simulink model "FSI_2DOF_SS_TF_Simulink"  (R2021a)
settings: Solver=FixedStepAuto  StartTime=0.0  StopTime=5  FixedStep=1e-4  RelTol=1e-3  EnableMultiTasking=on
undefined symbols (not defined in the file): A2, B2, bias_1, bias_2, C2, D2, den_2DOF_1, den_2DOF_2, F_1, F_2, is_1, is_2, num_2DOF_1, num_2DOF_2, omega_1, omega_2, phase_1, phase_2, t_1, t_2, v_10, v_20, x_10, x_20
settings Model: Creator=FilipKsica  LastModifiedBy=FilipKsica
settings SolverCC: AlgebraicLoopSolver=TrustRegion
settings DataIOCC: LimitDataPoints=on  ReturnWorkspaceOutputs=off
settings OptimizationCC: LifeSpan=inf
settings DebuggingCC: AllowSymbolicDim=off  SFUnexpectedBacktrackingDiag=warning  SFNoUnconditionalDefaultTransitionDiag=warning  SFExecutionAtInitializationDiag=none  SFMachineParentedDataDiag=warning  ArithmeticOperatorsInVariantConditions=warning
settings ModelReferenceCC: PropagateSignalLabelsOutOfModel=off
settings SFSimCC: SimUseLocalCustomCode=off  CustomCodeUndefinedFunction=UseInterfaceOnly
settings RTWCC: RTWUseLocalCustomCode=off
settings CodeAppCC: StateflowObjectComments=on
settings GRTTargetCC: TargetLangStandard=C89/C90 (ANSI)
settings ConfigComp: CovMetricSettings=dw  CovSaveCumulativeToWorkspaceVar=on  CovSaveSingleToWorkspaceVar=on  CovExternalEMLEnable=off

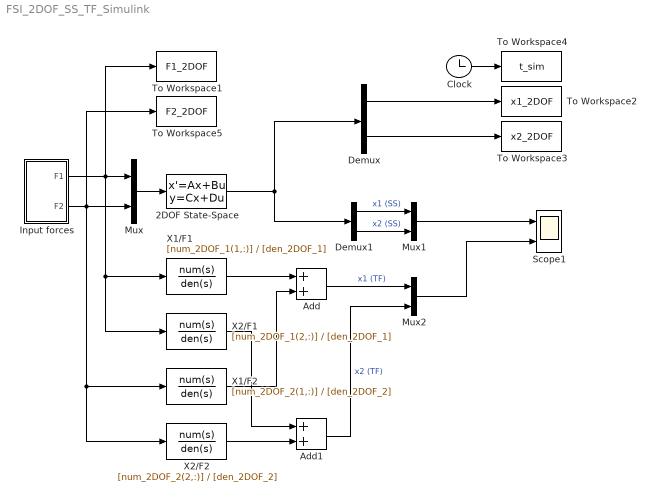
== system FSI_2DOF_SS_TF_Simulink ==
  2DOF State-Space : StateSpace  A=A2  B=B2  C=C2  D=D2  InitialCondition=[x_10 v_10 x_20 v_20]
  Add : Sum
  Add1 : Sum
  Clock : Clock
  Demux : Demux  Outputs=2
  Demux1 : Demux  Outputs=2
  Input forces : Subsystem
  Mux : Mux  Inputs=2
  Mux1 : Mux  Inputs=2
  Mux2 : Mux  Inputs=2
  Scope1 : Scope  NumInputPorts=2
  To Workspace1 : ToWorkspace  VariableName=F1_2DOF  SampleTime=-1
  To Workspace2 : ToWorkspace  VariableName=x1_2DOF  SampleTime=-1
  To Workspace3 : ToWorkspace  VariableName=x2_2DOF  SampleTime=-1
  To Workspace4 : ToWorkspace  VariableName=t_sim  SampleTime=-1
  To Workspace5 : ToWorkspace  VariableName=F2_2DOF  SampleTime=-1
  X1/F1 : TransferFcn  Numerator=[num_2DOF_1(1,:)]  Denominator=[den_2DOF_1]
  X1/F2 : TransferFcn  Numerator=[num_2DOF_2(1,:)]  Denominator=[den_2DOF_2]
  X2/F1 : TransferFcn  Numerator=[num_2DOF_1(2,:)]  Denominator=[den_2DOF_1]
  X2/F2 : TransferFcn  Numerator=[num_2DOF_2(2,:)]  Denominator=[den_2DOF_2]
  wires:
  Input forces/1(F1) -> To Workspace1/1, X2/F1/1, X1/F1/1, Mux/1
  Input forces/2("F2 ") -> To Workspace5/1, X2/F2/1, X1/F2/1, Mux/2
  Mux/1 -> 2DOF State-Space/1
  2DOF State-Space/1 -> Demux1/1, Demux/1
  Demux/1 -> To Workspace2/1
  Demux/2 -> To Workspace3/1
  Clock/1 -> To Workspace4/1
  Demux1/1 -> Mux1/1  "x1 (SS)"
  Demux1/2 -> Mux1/2  "x2 (SS)"
  Mux1/1 -> Scope1/1
  X1/F1/1 -> Add/1
  X1/F2/1 -> Add/2
  X2/F2/1 -> Add1/2
  X2/F1/1 -> Add1/1
  Add/1 -> Mux2/1  "x1 (TF)"
  Add1/1 -> Mux2/2  "x2 (TF)"
  Mux2/1 -> Scope1/2

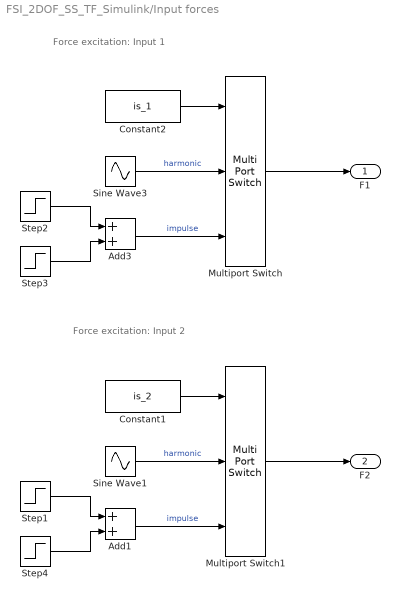
== system FSI_2DOF_SS_TF_Simulink/Input forces ==
  note: Force excitation: Input 1
  note: Force excitation: Input 2
  Add1 : Sum
  Add3 : Sum
  Constant1 : Constant  Value=is_2
  Constant2 : Constant  Value=is_1
  Multiport Switch : MultiPortSwitch  Inputs=2
  Multiport Switch1 : MultiPortSwitch  Inputs=2
  Sine Wave1 : Sin  Amplitude=F_2  Bias=bias_2  Frequency=omega_2  Phase=phase_2  SampleTime=0
  Sine Wave3 : Sin  Amplitude=F_1  Bias=bias_1  Frequency=omega_1  Phase=phase_1  SampleTime=0
  Step1 : Step  Time=0  After=F_2  SampleTime=0
  Step2 : Step  Time=0  After=F_1  SampleTime=0
  Step3 : Step  Time=t_1  After=-F_1  SampleTime=0
  Step4 : Step  Time=t_2  After=-F_2  SampleTime=0
  F1 : Outport  VectorParamsAs1DForOutWhenUnconnected=off
  "F2 " : Outport  Port=2  VectorParamsAs1DForOutWhenUnconnected=off
  wires:
  Step3/1 -> Add3/2
  Sine Wave3/1 -> Multiport Switch/2  "harmonic"
  Add3/1 -> Multiport Switch/3  "impulse"
  Step2/1 -> Add3/1
  Constant2/1 -> Multiport Switch/1
  Sine Wave1/1 -> Multiport Switch1/2  "harmonic"
  Add1/1 -> Multiport Switch1/3  "impulse"
  Constant1/1 -> Multiport Switch1/1
  Step1/1 -> Add1/1
  Step4/1 -> Add1/2
  Multiport Switch/1 -> F1/1
  Multiport Switch1/1 -> "F2 "/1
